simulink model "AXU5EV_Experiment_Encoder_Components"  (R2026b)
settings: Solver=VariableStepAuto
settings Model: Creator=lww  LastModifiedBy=lww

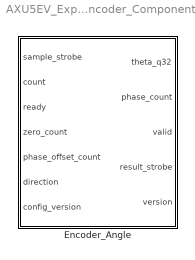
== system AXU5EV_Experiment_Encoder_Components ==
  Encoder_Angle : Subsystem  Description=Retained PR41 32-cycle serial modulo state and output registers. DSP electrical-scale Gain/Add blocks adapted to uint64 Q52, coefficient 943231700270, half 524288, shift20 -> signed64 Q32 radians. Test period30000 is unchanged.

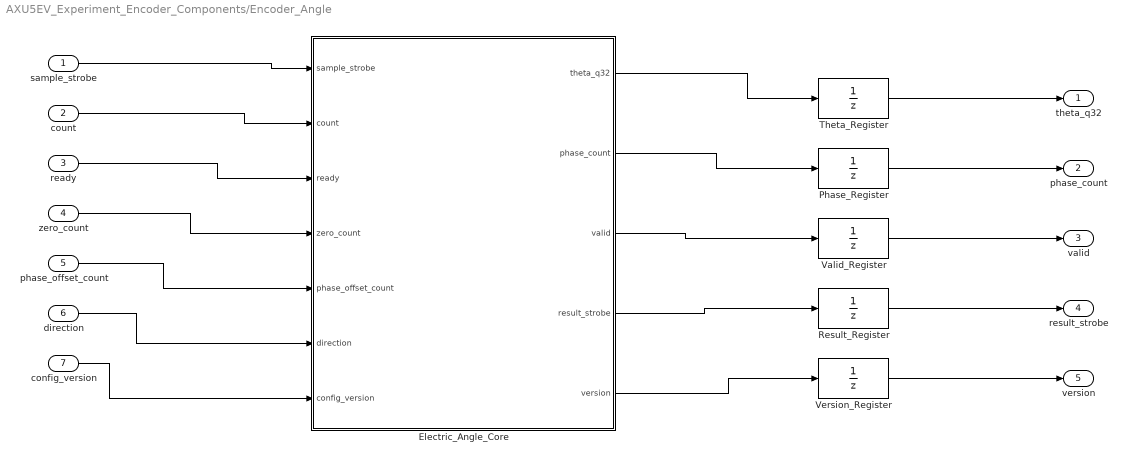
== system AXU5EV_Experiment_Encoder_Components/Encoder_Angle ==
  sample_strobe : Inport  OutDataTypeStr=boolean  SampleTime=2e-8
  count : Inport  Port=2  OutDataTypeStr=uint32  SampleTime=2e-8
  ready : Inport  Port=3  OutDataTypeStr=boolean  SampleTime=2e-8
  zero_count : Inport  Port=4  OutDataTypeStr=uint32  SampleTime=2e-8
  phase_offset_count : Inport  Port=5  OutDataTypeStr=uint16  SampleTime=2e-8
  direction : Inport  Port=6  OutDataTypeStr=boolean  SampleTime=2e-8
  config_version : Inport  Port=7  OutDataTypeStr=uint32  SampleTime=2e-8
  Electric_Angle_Core : Subsystem
  Phase_Register : UnitDelay  SampleTime=2e-8
  Result_Register : UnitDelay  SampleTime=2e-8
  Theta_Register : UnitDelay  SampleTime=2e-8
  Valid_Register : UnitDelay  SampleTime=2e-8
  Version_Register : UnitDelay  SampleTime=2e-8
  theta_q32 : Outport
  phase_count : Outport  Port=2
  valid : Outport  Port=3
  result_strobe : Outport  Port=4
  version : Outport  Port=5
  wires:
  Electric_Angle_Core/5(version) -> Version_Register/1
  Electric_Angle_Core/4(result_strobe) -> Result_Register/1
  Electric_Angle_Core/3(valid) -> Valid_Register/1
  Electric_Angle_Core/2(phase_count) -> Phase_Register/1
  Electric_Angle_Core/1(theta_q32) -> Theta_Register/1
  config_version/1 -> Electric_Angle_Core/7(config_version)
  direction/1 -> Electric_Angle_Core/6(direction)
  phase_offset_count/1 -> Electric_Angle_Core/5(phase_offset_count)
  zero_count/1 -> Electric_Angle_Core/4(zero_count)
  ready/1 -> Electric_Angle_Core/3(ready)
  count/1 -> Electric_Angle_Core/2(count)
  sample_strobe/1 -> Electric_Angle_Core/1(sample_strobe)
  Theta_Register/1 -> theta_q32/1
  Phase_Register/1 -> phase_count/1
  Valid_Register/1 -> valid/1
  Result_Register/1 -> result_strobe/1
  Version_Register/1 -> version/1

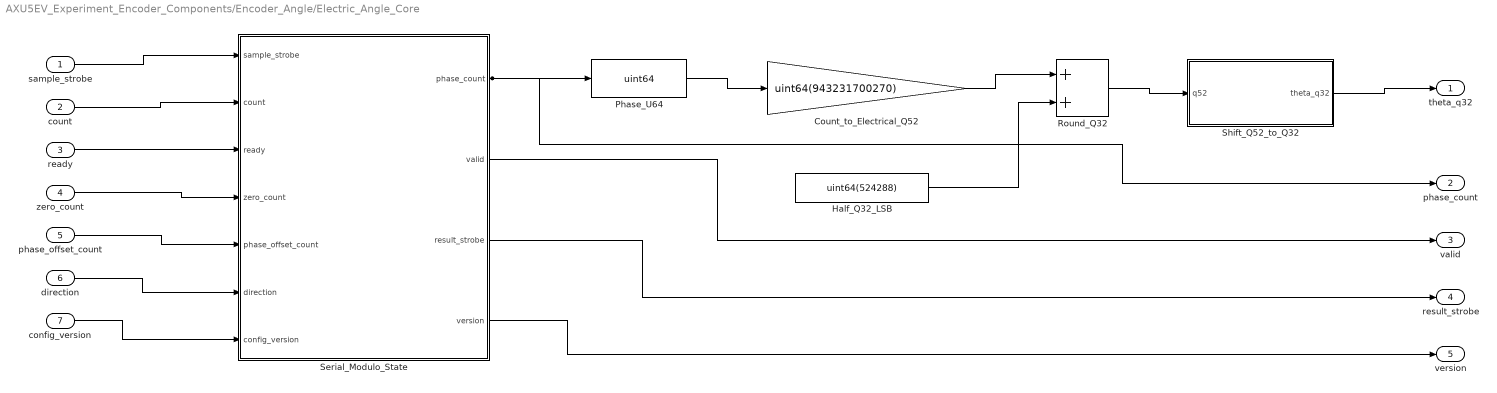
== system AXU5EV_Experiment_Encoder_Components/Encoder_Angle/Electric_Angle_Core ==
  sample_strobe : Inport
  count : Inport  Port=2
  ready : Inport  Port=3
  zero_count : Inport  Port=4
  phase_offset_count : Inport  Port=5
  direction : Inport  Port=6
  config_version : Inport  Port=7
  Count_to_Electrical_Q52 : Gain  Gain=uint64(943231700270)  ParamDataTypeStr=uint64  OutDataTypeStr=uint64
  Half_Q32_LSB : Constant  Value=uint64(524288)  OutDataTypeStr=uint64
  Phase_U64 : DataTypeConversion  OutDataTypeStr=uint64  SaturateOnIntegerOverflow=off  RndMeth=Floor
  Round_Q32 : Sum  OutDataTypeStr=uint64
  Serial_Modulo_State : MATLAB Function  TreatAsAtomicUnit=on
  Shift_Q52_to_Q32 : MATLAB Function  TreatAsAtomicUnit=on
  theta_q32 : Outport
  phase_count : Outport  Port=2
  valid : Outport  Port=3
  result_strobe : Outport  Port=4
  version : Outport  Port=5
  wires:
  Serial_Modulo_State/4(version) -> version/1
  Serial_Modulo_State/3(result_strobe) -> result_strobe/1
  Serial_Modulo_State/2(valid) -> valid/1
  Shift_Q52_to_Q32/1(theta_q32) -> theta_q32/1
  Round_Q32/1 -> Shift_Q52_to_Q32/1(q52)
  Half_Q32_LSB/1 -> Round_Q32/2
  Count_to_Electrical_Q52/1 -> Round_Q32/1
  Phase_U64/1 -> Count_to_Electrical_Q52/1
  Serial_Modulo_State/1(phase_count) -> phase_count/1, Phase_U64/1
  config_version/1 -> Serial_Modulo_State/7(config_version)
  direction/1 -> Serial_Modulo_State/6(direction)
  phase_offset_count/1 -> Serial_Modulo_State/5(phase_offset_count)
  zero_count/1 -> Serial_Modulo_State/4(zero_count)
  ready/1 -> Serial_Modulo_State/3(ready)
  count/1 -> Serial_Modulo_State/2(count)
  sample_strobe/1 -> Serial_Modulo_State/1(sample_strobe)

== matlab function AXU5EV_Experiment_Encoder_Components/Encoder_Angle/Electric_Angle_Core/Serial_Modulo_State ==
  data: sample_strobe input; phase_count output; count input; ready input; zero_count input; phase_offset_count input; direction input; config_version input; valid output; result_strobe output; version output
function [phase_count,valid,result_strobe,version]=f(sample_strobe,count,ready,zero_count,phase_offset_count,direction,config_version)
%#codegen
[phase_count,valid,result_strobe,version]=axu5ev_experiment_encoder_phase_serial(sample_strobe,count,ready,zero_count,phase_offset_count,direction,config_version);
end

== matlab function AXU5EV_Experiment_Encoder_Components/Encoder_Angle/Electric_Angle_Core/Shift_Q52_to_Q32 ==
  data: q52 input; theta_q32 output
function theta_q32=f(q52)
%#codegen
theta_q32=int64(bitshift(q52,-20));
end
